simulink model "ATOM_parking_chain"  (R2026a)
settings: Solver=ode4  StopTime=100  FixedStep=0.01
StopFcn:
  | % Put every new figure in the same MATLAB Figures window as a docked tab.
  | set(groot, 'defaultFigureWindowStyle', 'docked');
  | 
  | if exist('costmap_active', 'var') && ...
  |         exist('vehicle', 'var') && ...
  |         exist('parking_path', 'var') && ...
  |         ~isempty(parking_path)
  | 
  |     plotPlan(costmap_active, vehicle, parking_path);
  | 
  | else
  | 
  |     warning('No valid parking path is available for plotting.');
  | 
  | end
  | 
  | PlotControllerReferences( ...
  |     out.controller_reference_log);
  | 
  | PlotControllerTracking( ...
  |     out.controller_tracking_log);
undefined symbols (not defined in the file): lateral, longitudinal, stanley, vehicle
(part 3 of 11)

== matlab function ATOM_parking_chain/Parking Scenario1/freespace_planner/freespacePlanner ==
  settings: updateMethod=DISCRETE
  data: x output; y output; z output; qx output; qy output; qz output; qw output; longitudinal_velocity_mps output; lateral_velocity_mps output; acceleration_mps2 output; heading_rate_rps output; front_wheel_angle_rad output; rear_wheel_angle_rad output; start_pose input; goal_pose input; veh input; costmap input Bus: OccupancyGridBus; segment_request input; segment_count output
function [x,y,z,qx,qy,qz,qw, longitudinal_velocity_mps, ...
          lateral_velocity_mps, acceleration_mps2, ...
          heading_rate_rps, front_wheel_angle_rad, ...
          rear_wheel_angle_rad, segment_count] = ...
          freespacePlanner( ...
          start_pose, goal_pose, veh, costmap, segment_request)
%FREESPACEPLANNER
% Run Hybrid A* once and publish the requested gear segment.

N = 100;

coder.extrinsic('planParkingTrajectory');

persistent T active_segment cached_segment_count

% Initial planning call.
if isempty(T)

    T = zeros(N,13);

    active_segment = 1.0;
    cached_segment_count = 0.0;

    % reset_plan=true causes Hybrid A* to compute a new complete path.
    [T, cached_segment_count] = planParkingTrajectory( ...
        costmap, start_pose, goal_pose, veh, 1.0, true);
end

% Convert the external request into a valid segment number.
requested_segment = round(double(segment_request));
requested_segment = max(1.0, requested_segment);

if cached_segment_count > 0
    requested_segment = min( ...
        requested_segment, cached_segment_count);
else
    requested_segment = 1.0;
end

% Change the published segment without running Hybrid A* again.
if requested_segment ~= active_segment && ...
        cached_segment_count > 0

    [T, cached_segment_count] = planParkingTrajectory( ...
        costmap, start_pose, goal_pose, veh, ...
        requested_segment, false);

    active_segment = requested_segment;
end

segment_count = cached_segment_count;

% Publish the selected segment through the existing trajectory signals.
x  = T(:,1);
y  = T(:,2);
z  = T(:,3);

qx = T(:,4);
qy = T(:,5);
qz = T(:,6);
qw = T(:,7);

longitudinal_velocity_mps = T(:,8);
lateral_velocity_mps      = T(:,9);
acceleration_mps2         = T(:,10);
heading_rate_rps          = T(:,11);
front_wheel_angle_rad     = T(:,12);
rear_wheel_angle_rad      = T(:,13);
end

== matlab function ATOM_parking_chain/Plot vehicle2/Plot Vehicle Rear reference frame ==
  settings: updateMethod=DISCRETE
  data: kinematic input Bus: KinematicStateBus; steer_front input double; steer_rear input double; veh input; traj input; costmap input
   function plotVehicleRear(kinematic, steer_front, steer_rear, veh, traj, costmap)
  coder.extrinsic('imagesc','colormap','evalin');
%% Vehicle parameters

L  = veh(3);
track = veh(4);

front_overhang = veh(5);
rear_overhang  = veh(6);
left_overhang = veh(7);
right_overhang = veh(8);

vehicle_length  = L + front_overhang + rear_overhang;
vehicle_width = track + left_overhang + right_overhang;

wheel_width = veh(2);
wheel_radius = veh(1);

%% Reference trajectory

x_ref = evalin('base', 'parking_path(:,1)');
y_ref = evalin('base', 'parking_path(:,2)');


%% Current kinematic state

x = kinematic.pose.position.x;
y = kinematic.pose.position.y;

qz = kinematic.pose.orientation.z;
qw = kinematic.pose.orientation.w;

yaw = 2*atan2(qz,qw);

vx = kinematic.twist.linear.x;

steer_front = steer_front;
steer_rear = steer_rear;

%% Position and orientation vehicle body

vehicle_body = [L+front_overhang vehicle_width/2;
                L+front_overhang -vehicle_width/2;
                -rear_overhang -vehicle_width/2;
                -rear_overhang vehicle_width/2;
                L+front_overhang vehicle_width/2];

R_body = [ cos(yaw) -sin(yaw)
    sin(yaw)  cos(yaw) ];

body_world = (R_body*vehicle_body')';

body_world(:,1)=body_world(:,1)+x;
body_world(:,2)=body_world(:,2)+y;


%% Position and orientation wheels

wheel_body = [wheel_radius  wheel_width/2
                wheel_radius -wheel_width/2
                -wheel_radius -wheel_width/2
                -wheel_radius  wheel_width/2
                wheel_radius  wheel_width/2];

FL = [L  track/2];
FR = [L -track/2];
RL = [0  track/2];
RR = [0 -track/2];

centers = [FL;
    FR;
    RL;
    RR];

centers = (R_body*centers')';

centers(:,1) = centers(:,1)+x;
centers(:,2) = centers(:,2)+y;

wheelFL = transformWheel(centers(1,:),steer_front,yaw,wheel_body);
wheelFR = transformWheel(centers(2,:),steer_front,yaw,wheel_body);
wheelRL = transformWheel(centers(3,:),steer_rear,yaw,wheel_body);
wheelRR = transformWheel(centers(4,:),steer_rear,yaw,wheel_body);



persistent hFig
persistent ax
persistent hBody
persistent hWheelFL
persistent hWheelFR
persistent hWheelRL
persistent hWheelRR
persistent hTrajectory
persistent TrajX
persistent TrajY
persistent hRefTraj 


if isempty(hBody)
    hFig = figure(20);
    clf

    ax = axes(hFig);

    hold(ax,'on')
    axis(ax,'equal')
    grid(ax,'on')


    xlabel(ax,'x [m]')
    ylabel(ax,'y [m]')

    % --- obstacles: the same costmap the planner used ---
    res = double(costmap.info.resolution);
    W   = double(costmap.info.width);
    H   = double(costmap.info.height);
    ox  = double(costmap.info.origin.position.x);
    oy  = double(costmap.info.origin.position.y);
    g   = double(costmap.data);
    imagesc(ax, ox+(0:W-1)*res, oy+(0:H-1)*res, g, 'AlphaData', (g>=100)*0.55);
    colormap(ax, [1 1 1; 0.85 0.25 0.25]);
    set(ax, 'YDir','normal', 'Layer','top');

    hBody = plot(body_world(:,1),...
        body_world(:,2),...
        'k','LineWidth',2);

    hWheelFL = plot(wheelFL(:,1),...
        wheelFL(:,2),...
        'r','LineWidth',2);

    hWheelFR = plot(wheelFR(:,1),...
        wheelFR(:,2),...
        'r','LineWidth',2);

    hWheelRL = plot(wheelRL(:,1),...
        wheelRL(:,2),...
        'b','LineWidth',2);

    hWheelRR = plot(wheelRR(:,1),...
        wheelRR(:,2),...
        'b','LineWidth',2);

    TrajX = x;
    TrajY = y;

   hTrajectory = plot(TrajX, TrajY, 'g', 'LineWidth', 3);
   hRefTraj    = plot(x_ref, y_ref, 'b', 'LineWidth', 1);

else

    set(hBody,...
        'XData',body_world(:,1),...
        'YData',body_world(:,2));

    set(hWheelFL,...
        'XData',wheelFL(:,1),...
        'YData',wheelFL(:,2));

    set(hWheelFR,...
        'XData',wheelFR(:,1),...
        'YData',wheelFR(:,2));

    set(hWheelRL,...
        'XData',wheelRL(:,1),...
        'YData',wheelRL(:,2));

    set(hWheelRR,...
        'XData',wheelRR(:,1),...
        'YData',wheelRR(:,2));

    TrajX(end+1) = x;
    TrajY(end+1) = y;

 
    set(hTrajectory,...
        'XData',TrajX,...
        'YData',TrajY);

    set(hRefTraj,...
        'XData',x_ref,...
        'YData',y_ref);

end

   xlim(ax, [-16 16])
   ylim(ax, [-14 14])

% xlim([-20 20])
% ylim([-20 20])

drawnow limitrate


end

== matlab function ATOM_parking_chain/Plot vehicle2/Plot vehicle Front reference frame ==
  settings: updateMethod=DISCRETE
  data: kinematic input Bus: KinematicStateBus; steer_front input double; steer_rear input double; veh input; traj input
function plotVehicleFront(kinematic, steer_front, steer_rear, veh, traj)

%% Vehicle parameters

L  = veh(3);
track = veh(4);

front_overhang = veh(5);
rear_overhang  = veh(6);
left_overhang = veh(7);
right_overhang = veh(8);

vehicle_length  = L + front_overhang + rear_overhang;
vehicle_width = track + left_overhang + right_overhang;

wheel_width = veh(2);
wheel_radius = veh(1);

%% Reference trajectory

x_ref = traj.pose.position.x;
y_ref = traj.pose.position.y;

yaw_ref = zeros(length(x_ref),1);


for i=1:length(x_ref)

    yaw_ref(i)=2*atan2(...
        traj.pose.orientation.qz(i),...
        traj.pose.orientation.qw(i));
end


%% Current kinematic state

x = kinematic.pose.position.x;
y = kinematic.pose.position.y;

qz = kinematic.pose.orientation.z;
qw = kinematic.pose.orientation.w;

yaw = 2*atan2(qz,qw);

vx = kinematic.twist.linear.x;

steer_front = steer_front;
steer_rear = steer_rear;

%% Position and orientation vehicle body

vehicle_body = [front_overhang vehicle_width/2;
                front_overhang -vehicle_width/2;
                -L-rear_overhang -vehicle_width/2;
                -L-rear_overhang vehicle_width/2;
                front_overhang vehicle_width/2];

R_body = [ cos(yaw) -sin(yaw)
    sin(yaw)  cos(yaw) ];

body_world = (R_body*vehicle_body')';

body_world(:,1)=body_world(:,1)+x;
body_world(:,2)=body_world(:,2)+y;


%% Position and orientation wheels

wheel_body = [wheel_radius  wheel_width/2
                wheel_radius -wheel_width/2
                -wheel_radius -wheel_width/2
                -wheel_radius  wheel_width/2
                wheel_radius  wheel_width/2];

FL = [0  track/2];
FR = [0 -track/2];
RL = [-L  track/2];
RR = [-L -track/2];

centers = [FL;
    FR;
    RL;
    RR];

centers = (R_body*centers')';

centers(:,1) = centers(:,1)+x;
centers(:,2) = centers(:,2)+y;

wheelFL = transformWheel(centers(1,:),steer_front,yaw,wheel_body);
wheelFR = transformWheel(centers(2,:),steer_front,yaw,wheel_body);
wheelRL = transformWheel(centers(3,:),steer_rear,yaw,wheel_body);
wheelRR = transformWheel(centers(4,:),steer_rear,yaw,wheel_body);



persistent hFig
persistent ax
persistent hBody
persistent hWheelFL
persistent hWheelFR
persistent hWheelRL
persistent hWheelRR
persistent hTrajectory
persistent TrajX
persistent TrajY
persistent hRefTraj 
persistent hArrow


if isempty(hBody)
    hFig = figure(13);
    clf

    ax = axes(hFig);

    hold(ax,'on')
    axis(ax,'equal')
    grid(ax,'on')


    xlabel(ax,'x [m]')
    ylabel(ax,'y [m]')

    hBody = plot(body_world(:,1),...
        body_world(:,2),...
        'k','LineWidth',2);

    hWheelFL = plot(wheelFL(:,1),...
        wheelFL(:,2),...
        'r','LineWidth',2);

    hWheelFR = plot(wheelFR(:,1),...
        wheelFR(:,2),...
        'r','LineWidth',2);

    hWheelRL = plot(wheelRL(:,1),...
        wheelRL(:,2),...
        'b','LineWidth',2);

    hWheelRR = plot(wheelRR(:,1),...
        wheelRR(:,2),...
        'b','LineWidth',2);

    TrajX = x;
    TrajY = y;

    hTrajectory = plot(TrajX,...
                       TrajY,...
                       'g','LineWidth',1);

    hRefTraj=plot(x_ref,y_ref,'b','LineWidth',2);

    step=5;

    hArrow=quiver(...
        x_ref(1:step:end),...
        y_ref(1:step:end),...
        cos(yaw_ref(1:step:end)),...
        sin(yaw_ref(1:step:end)),...
        0.5,...
        'r');

else

    set(hBody,...
        'XData',body_world(:,1),...
        'YData',body_world(:,2));

    set(hWheelFL,...
        'XData',wheelFL(:,1),...
        'YData',wheelFL(:,2));

    set(hWheelFR,...
        'XData',wheelFR(:,1),...
        'YData',wheelFR(:,2));

    set(hWheelRL,...
        'XData',wheelRL(:,1),...
        'YData',wheelRL(:,2));

    set(hWheelRR,...
        'XData',wheelRR(:,1),...
        'YData',wheelRR(:,2));

    TrajX(end+1) = x;
    TrajY(end+1) = y;

 
    set(hTrajectory,...
        'XData',TrajX,...
        'YData',TrajY);

    set(hRefTraj,...
        'XData',x_ref,...
        'YData',y_ref);

    

end

margin = 12;
xlim(ax, [x-margin x+margin])
ylim(ax, [y-margin y+margin])

% xlim([-20 20])
% ylim([-20 20])

drawnow limitrate


end

== matlab function ATOM_parking_chain/Plot vehicle2/RearToFrontOdometry ==
  data: rear_pose input Bus: KinematicStateBus; front_pose output Bus: KinematicStateBus; wheel_base input
function front_pose = RearToFrontOdometry( ...
    rear_pose,...
    wheel_base)


front_pose = rear_pose;


qx = rear_pose.pose.orientation.x;
qy = rear_pose.pose.orientation.y;
qz = rear_pose.pose.orientation.z;
qw = rear_pose.pose.orientation.w;


yaw = QuaternionToYaw(qx,qy,qz,qw);



front_pose.pose.position.x = ...
    rear_pose.pose.position.x + ...
    wheel_base*cos(yaw);


front_pose.pose.position.y = ...
    rear_pose.pose.position.y + ...
    wheel_base*sin(yaw);


front_pose.pose.position.z = ...
    rear_pose.pose.position.z;



% orientation unchanged

front_pose.pose.orientation = ...
    rear_pose.pose.orientation;


% Linear velocity referred to front axle

front_pose.twist.linear.x = rear_pose.twist.linear.x ...
    - rear_pose.twist.angular.z ...
    * wheel_base*sin(yaw);


front_pose.twist.linear.y = rear_pose.twist.linear.y ...
    + rear_pose.twist.angular.z ...
    * wheel_base*cos(yaw);


front_pose.twist.linear.z = rear_pose.twist.linear.z;


end

== matlab function ATOM_parking_chain/Plot vehicle2/SetStanleyTrajectory/Resample Trajectory ==
  data: trajectory_in input Bus: TrajectoryDataBus; trajectory_out output Bus: TrajectoryDataBus; resample_interval_dist input; nearest_seg_idx input; ego_offset_to_segment input
function trajectory_out = resampleTrajectoryByDistance( ...
    trajectory_in, ...
    resample_interval_dist, ...
    nearest_seg_idx, ...
    ego_offset_to_segment)


%% ============================================================
% RESAMPLE TRAJECTORY BY ARC LENGTH
%
% Equivalent to:
%
% MPCUtils::resampleMPCTrajectoryByDistance()
%
% Adapted for Stanley controller.
%
% Unlike MPC:
% - no MPCTrajectory conversion
% - no curvature resampling
% - no optimization variables
%
% The trajectory is directly interpolated in arc length.
%
% ATTENTION:
% 
% Resampling is not actuated in Simulink since in/out buses present fixed sizes.
% See NOTE at the end of this function.
%
% =============================================================


% N = length(trajectory_in.pose.position.x);
% 
% 
% if N < 2
% 
%     trajectory_out = trajectory_in;
%     return
% 
% end
% 
% 
% 
% %% ============================================================
% % Compute arc length
% % =============================================================
% 
% x = trajectory_in.pose.position.x;
% y = trajectory_in.pose.position.y;
% 
% 
% arc_length = zeros(N,1);
% 
% 
% for i = 2:N
% 
%     dx = x(i)-x(i-1);
%     dy = y(i)-y(i-1);
% 
%     arc_length(i)= ...
%         arc_length(i-1)+sqrt(dx^2+dy^2);
% 
% end
% 
% 
% 
% if isempty(arc_length)
% 
%     trajectory_out = trajectory_in;
%     return
% 
% end
% 
% 
% 
% %% ============================================================
% % Ego position along trajectory
% %
% % Equivalent to:
% %
% % input_arclength(nearest_seg_idx)
% % + ego_offset_to_segment
% %
% % =============================================================
% 
% 
% ego_s = arc_length(nearest_seg_idx) ...
%         + ego_offset_to_segment;
% 
% 
% ego_s = min(max(ego_s,0),arc_length(end));
% 
% 
% 
% %% ============================================================
% % Generate resampling points
% %
% % Same strategy as Autoware:
% % - backward from ego
% % - forward from ego
% %
% % =============================================================
% 
% 
% output_s = [];
% 
% 
% % backward direction
% 
% s = ego_s;
% 
% while s >= 0
% 
%     output_s = [s output_s]; %#ok<AGROW>
% 
%     s = s - resample_interval_dist;
% 
% end
% 
% 
% 
% % forward direction
% 
% s = ego_s + resample_interval_dist;
% 
% 
% while s < arc_length(end)
% 
%     output_s(end+1)=s; % #ok<AGROW>
% 
%     s = s + resample_interval_dist;
% 
% end
% 
% 
% 
% %% ============================================================
% % Interpolation
% % =============================================================
% 
% 
% x_new = interp1( ...
%     arc_length,...
%     x,...
%     output_s,...
%     'linear');
% 
% 
% 
% y_new = interp1( ...
%     arc_length,...
%     y,...
%     output_s,...
%     'linear');
% 
% 
% 
% z = trajectory_in.pose.position.z;
% 
% z_new = interp1( ...
%     arc_length,...
%     z,...
%     output_s,...
%     'linear');
% 
% 
% 
% %% ============================================================
% % Quaternion / yaw interpolation
% %
% % Stanley works with yaw.
% % Therefore interpolate yaw and rebuild quaternion.
% %
% % =============================================================
% 
% 
% yaw = QuaternionToYaw( ...
%     trajectory_in.pose.orientation.qx,...
%     trajectory_in.pose.orientation.qy,...
%     trajectory_in.pose.orientation.qz,...
%     trajectory_in.pose.orientation.qw);
% 
% 
% 
% % avoid discontinuity
% 
% yaw = unwrap(yaw);
% 
% 
% 
% yaw_new = interp1( ...
%     arc_length,...
%     yaw,...
%     output_s,...
%     'linear');
% 
% 
% 
% %% ============================================================
% % Velocity interpolation
% %
% % Autoware uses linear interpolation
% % =============================================================
% 
% 
% vel_new = interp1( ...
%     arc_length,...
%     trajectory_in.longitudinal_velocity_mps,...
%     output_s,...
%     'linear');
% 
% 
% 
% lat_vel_new = interp1( ...
%     arc_length,...
%     trajectory_in.lateral_velocity_mps,...
%     output_s,...
%     'linear');
% 
% 
% 
% acc_new = interp1( ...
%     arc_length,...
%     trajectory_in.acceleration_mps2,...
%     output_s,...
%     'linear');
% 
% 
% 
% %% ============================================================
% % Build output structure
% % =============================================================
% 
% 
% M = length(output_s);
% 
% 
% trajectory_out.pose.position.x = x_new;
% trajectory_out.pose.position.y = y_new;
% trajectory_out.pose.position.z = z_new;
% 
% 
% 
% [qx,qy,qz,qw] = yawToQuaternion(yaw_new);
% 
% 
% 
% trajectory_out.pose.orientation.qx = qx;
% trajectory_out.pose.orientation.qy = qy;
% trajectory_out.pose.orientation.qz = qz;
% trajectory_out.pose.orientation.qw = qw;
% 
% 
% 
% trajectory_out.longitudinal_velocity_mps = vel_new;
% 
% trajectory_out.lateral_velocity_mps = lat_vel_new;
% 
% trajectory_out.acceleration_mps2 = acc_new;
% 
% 
% 
% % steering values are kept
% 
% trajectory_out.front_wheel_angle_rad = ...
%     interp1( ...
%     arc_length,...
%     trajectory_in.front_wheel_angle_rad,...
%     output_s,...
%     'linear');
% 
% 
% trajectory_out.rear_wheel_angle_rad = ...
%     interp1( ...
%     arc_length,...
%     trajectory_in.rear_wheel_angle_rad,...
%     output_s,...
%     'linear');
% 
% 


%% ============================================================
% NOTE (Simulink Implementation)
%
% The trajectory resampling algorithm reported above is equivalent
% to the implementation adopted by Autoware.
%
% However, the main objective of the present work is the development
% and validation of the 4WS Stanley Controller rather than the
% trajectory preprocessing module.
%
% Since Simulink requires fixed-size bus signals, the resampled
% trajectory is not generated in the simulation model.
%
% The original input trajectory is therefore directly propagated to
% the controller, preserving its fixed dimension and avoiding the
% introduction of variable-length signals.
%
% Consequently, the following assignment overwrites the resampled
% trajectory computed above.
%
% ============================================================

trajectory_out = trajectory_in;

end

== matlab function ATOM_parking_chain/Plot vehicle2/SetStanleyTrajectory/calcLongOffsetToSegment ==
  data: seg_idx input; ego_pose input; trajectory input Bus: TrajectoryDataBus; ego_offset_to_segment output
function ego_offset_to_segment = calcLongOffsetToSegment(seg_idx, ego_pose, trajectory)

ego_offset_to_segment = calcLongitudinalOffsetToSegment(trajectory, seg_idx, ego_pose);

end

== matlab function ATOM_parking_chain/Plot vehicle2/SetStanleyTrajectory/findFirstNearestSegmentIndexWithSoftConstraints ==
  data: trajectory input; dist_threshold input; yaw_threshold input; nearest_seg_idx output; pose input
function nearest_seg_idx = findNearestSegmentIndexWithSoftConstraints( ...
    trajectory, dist_threshold, yaw_threshold, pose)


%% Step 1:
% Find nearest point index

nearest_idx = findFirstNearestIndexWithSoftConstraints( ...
    trajectory, ...
    pose, ...
    dist_threshold, ...
    yaw_threshold);


N = length(trajectory.pose.position.x);


%% Step 2:
% Convert point index into segment index

% First point
if nearest_idx == 1

    nearest_seg_idx = 1;
    return

end


% Last point
if nearest_idx == N

    nearest_seg_idx = N-1;
    return

end



%% Step 3:
% Determine whether ego lies before or after nearest point
%
% Equivalent to Autoware:
%
% signed_length =
% calcLongitudinalOffsetToSegment(points,
%                                 nearest_idx,
%                                 pose.position)


signed_length = calcLongitudinalOffsetToSegment( ...
    trajectory,...
    nearest_idx,...
    pose);



%% Step 4:
% Choose segment

if signed_length <= 0

    % ego is before nearest point
    %
    % Autoware:
    % return nearest_idx - 1;

    nearest_seg_idx = nearest_idx - 1;


else

    % ego is after nearest point
    %
    % Autoware:
    % return nearest_idx;

    nearest_seg_idx = nearest_idx;

end


end

== matlab function ATOM_parking_chain/Subsystem1/MATLAB Function ==
  data: a_cmd_previous input; a_cmd_history output
function a_cmd_history = ...
    accelerationCommandHistory(a_cmd_previous)

persistent history

if isempty(history)
    history = repmat(a_cmd_previous,3,1);
else
    history = ...
        [history(2:end);a_cmd_previous];
end

a_cmd_history = history;
end

== matlab function ATOM_parking_chain/Subsystem1/parkingLongitudinalController ==
  data: tx input; a_cmd output; ty input; tvx input; tax input; s_now input; vx input; longitudinal_mode input; a_ref_out output; v_ref_out output
function [a_cmd,a_ref_out,v_ref_out] = parkingLongitudinalController( ...
    tx, ty, tvx, tax, s_now, vx, longitudinal_mode)
%#codegen
%
% Independent longitudinal parking controller.
%
% Inputs:
%   tx, ty  : trajectory position arrays
%   tvx     : signed velocity reference array
%   tax     : signed acceleration feedforward array
%   s_now   : current progress along the trajectory
%   vx      : measured longitudinal velocity
%   longitudinal_mode:
%             0 = normal profile tracking
%             1 = terminal creep
%             2 = stop
%
% Output:
%   a_cmd   : commanded longitudinal acceleration

N = 100;

% Normal velocity-tracking gain.
Kp = 1.0;

% Stronger gain used only when stopping at a segment endpoint.
% With the 1 m/s^2 command limit, this requests maximum braking whenever
% the speed magnitude is greater than or equal to 0.20 m/s.
Kp_stop = 5.0;

% Existing velocity-smoother longitudinal acceleration limit.
a_cmd_limit = 1.0;

terminal_creep_speed = 0.05;

%% Construct trajectory arc length

s = zeros(N,1);

for k = 2:N
    s(k) = s(k-1) + hypot( ...
        tx(k)-tx(k-1), ...
        ty(k)-ty(k-1));
end

%% Read the feedforward references at the current progress

v_ref = lookupS(s,tvx,s_now);
a_ref = lookupS(s,tax,s_now);

%% Determine the forward or reverse direction

gear = 1.0;

for k = 1:N
    if abs(tvx(k)) > 1e-6
        gear = sign(tvx(k));
        break;
    end
end

%% Apply the maneuver-supervisor mode
%% Apply the maneuver-supervisor mode

% Use the normal tracking gain unless stop mode selects the stronger gain.
Kp_active = Kp;

if longitudinal_mode == 2.0

    % Stop mode.
    % Drive the measured velocity firmly toward zero.
    v_ref = 0.0;
    a_ref = 0.0;
    Kp_active = Kp_stop;

elseif longitudinal_mode == 1.0

    % Very slow endpoint correction.
    v_ref = gear*terminal_creep_speed;
    a_ref = 0.0;

end

% Acceleration reference currently selected at the vehicle's progress.
a_ref_out = a_ref;
v_ref_out = v_ref;
%% Feedforward plus velocity-error correction

%% Feedforward plus velocity-error correction

speed_error = v_ref - vx;

% Express the measured and reference velocities in the direction of the
% current segment. Positive means movement in the intended gear direction.
speed_in_gear = gear * vx;
reference_speed_in_gear = gear * v_ref;
feedforward_in_gear = gear * a_ref;

% A negative feedforward value means braking.
%
% Apply braking feedforward only while the vehicle is moving faster than
% its reference. Once the vehicle is at or below the reference speed,
% remove the braking feedforward and let the velocity feedback correct it.
%
% This also prevents the controller from intentionally accelerating the
% vehicle in the opposite direction before the segment manager authorizes
% a gear change.
a_feedforward = a_ref;

if feedforward_in_gear < 0.0 && ...
        speed_in_gear <= reference_speed_in_gear

    a_feedforward = 0.0;

end

a_unsaturated = ...
    a_feedforward + Kp_active*speed_error;

a_cmd = max( ...
    -a_cmd_limit, ...
    min(a_cmd_limit,a_unsaturated));

end

%--------------------------------------------------------------------------
function value = lookupS(sv,vv,s_query)
% Linear interpolation of a trajectory quantity by path distance.

n = numel(sv);
value = vv(n);

if s_query <= sv(1)
    value = vv(1);
    return;
end

if s_query >= sv(n)
    return;
end

for k = 1:n-1

    if s_query <= sv(k+1)

        ds = sv(k+1)-sv(k);

        if ds < 1e-12
            value = vv(k+1);
        else
            ratio = (s_query-sv(k))/ds;
            value = vv(k) + ratio*(vv(k+1)-vv(k));
        end

        return;
    end
end

end
